simulink model "TCLab_Test_PIL"  (R2026a)
settings: Solver=FixedStepDiscrete  StopTime=t_final  FixedStep=Ts
InitFcn:
  | A8_init_TCLab_SIMC
undefined symbols (not defined in the file): den_Gp_d, dspblkCoreblockFVToolHelper, gcbh, N_delay, num_Gp_d, T_amb, T_ref, Ts
settings Model: SILPILSystemUnderTest=refmodels  Creator=jguerrero  LastModifiedBy=jordy

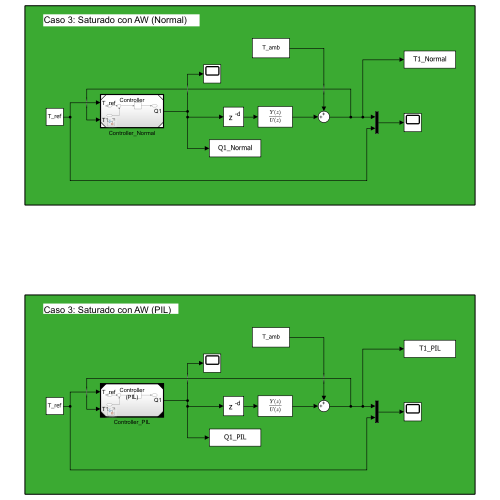
[thumbnail: Simulink's stored preview of the top-level diagram]
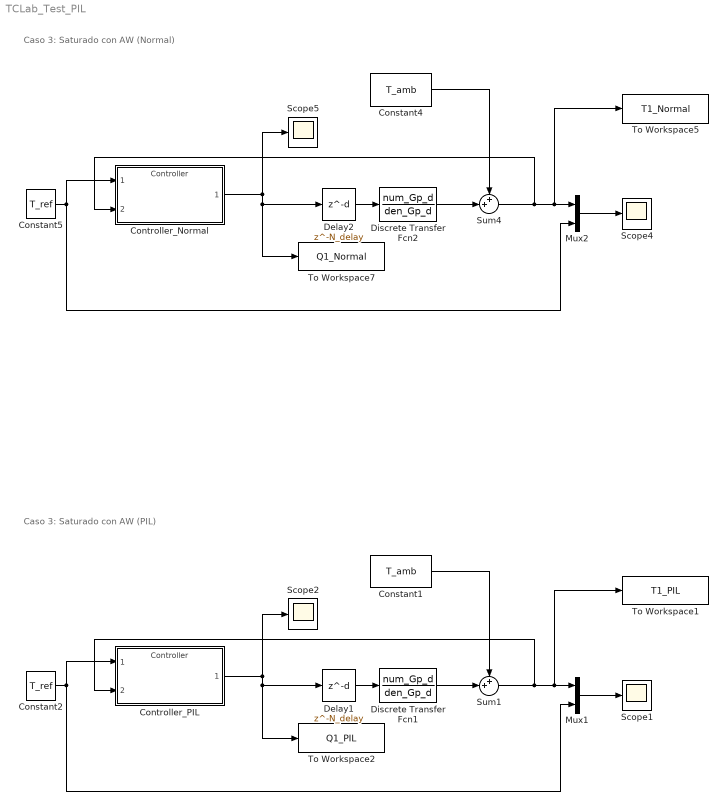
== system TCLab_Test_PIL ==
  note: Caso 3: Saturado con AW (Normal)
  note: Caso 3: Saturado con AW (PIL)
  Constant1 : Constant  Value=T_amb  OutDataTypeStr=single  SampleTime=Ts
  Constant2 : Constant  Value=T_ref  OutDataTypeStr=single  SampleTime=Ts
  Constant4 : Constant  Value=T_amb  OutDataTypeStr=single  SampleTime=Ts
  Constant5 : Constant  Value=T_ref  OutDataTypeStr=single  SampleTime=Ts
  Controller_Normal : ModelReference  ModelNameDialog=Controller  SimulationMode=Normal  ModelReferenceVersion=1.20
  Controller_PIL : ModelReference  ModelNameDialog=Controller  SimulationMode=Processor-in-the-loop (PIL)  ModelReferenceVersion=1.20
  Delay1 : Delay  DelayLength=N_delay  SampleTime=Ts
  Delay2 : Delay  DelayLength=N_delay  SampleTime=Ts
  Discrete Transfer Fcn1 : DiscreteTransferFcn  LoadFcn=dspblkCoreblockFVToolHelper(gcbh,'load');  Numerator=num_Gp_d  Denominator=den_Gp_d
      settings: CopyFcn=dspblkCoreblockFVToolHelper(gcbh,'copy');  DeleteFcn=dspblkCoreblockFVToolHelper(gcbh,'close');  ModelCloseFcn=dspblkCoreblockFVToolHelper(gcbh,'close');  PreSaveFcn=dspblkCoreblockFVToolHelper(gcbh,'presave');  PostSaveFcn=dspblkCoreblockFVToolHelper(gcbh,'postsave');  CloseFcn=dspblkCoreblockFVToolHelper(gcbh,'close');
  Discrete Transfer Fcn2 : DiscreteTransferFcn  LoadFcn=dspblkCoreblockFVToolHelper(gcbh,'load');  Numerator=num_Gp_d  Denominator=den_Gp_d
      settings: CopyFcn=dspblkCoreblockFVToolHelper(gcbh,'copy');  DeleteFcn=dspblkCoreblockFVToolHelper(gcbh,'close');  ModelCloseFcn=dspblkCoreblockFVToolHelper(gcbh,'close');  PreSaveFcn=dspblkCoreblockFVToolHelper(gcbh,'presave');  PostSaveFcn=dspblkCoreblockFVToolHelper(gcbh,'postsave');  CloseFcn=dspblkCoreblockFVToolHelper(gcbh,'close');
  Mux1 : Mux  Inputs=2
  Mux2 : Mux  Inputs=2
  Scope{1..2,4..5} (4 alike) : Scope
      Scope1 settings: ActiveDisplayYMinimum=20.625  ActiveDisplayYMaximum=64.375
      Scope2 settings: ActiveDisplayYMinimum=27.921311930843586  ActiveDisplayYMaximum=96.897632007684052
      Scope4 settings: ActiveDisplayYMinimum=20.625  ActiveDisplayYMaximum=64.375  DataLoggingVariableName=ScopeData4
      Scope5 settings: ActiveDisplayYMinimum=27.921311930843586  ActiveDisplayYMaximum=96.897632007684052  DataLoggingVariableName=ScopeData5
  Sum1 : Sum  Inputs=++|  OutDataTypeStr=single  AccumDataTypeStr=single
  Sum4 : Sum  Inputs=++|  OutDataTypeStr=single  AccumDataTypeStr=single
  To Workspace1 : ToWorkspace  VariableName=T1_PIL  SaveFormat=Timeseries  SampleTime=-1
  To Workspace2 : ToWorkspace  VariableName=Q1_PIL  SaveFormat=Timeseries  SampleTime=-1
  To Workspace5 : ToWorkspace  VariableName=T1_Normal  SaveFormat=Timeseries  SampleTime=-1
  To Workspace7 : ToWorkspace  VariableName=Q1_Normal  SaveFormat=Timeseries  SampleTime=-1
  wires:
  Constant4/1 -> Sum4/1
  Sum4/1 -> Controller_Normal/2, Mux2/1, To Workspace5/1
  Delay2/1 -> Discrete Transfer Fcn2/1
  Discrete Transfer Fcn2/1 -> Sum4/2
  Mux2/1 -> Scope4/1
  Constant5/1 -> Controller_Normal/1, Mux2/2
  Controller_Normal/1 -> To Workspace7/1, Delay2/1, Scope5/1
  Mux1/1 -> Scope1/1
  Constant1/1 -> Sum1/1
  Delay1/1 -> Discrete Transfer Fcn1/1
  Controller_PIL/1 -> To Workspace2/1, Delay1/1, Scope2/1
  Constant2/1 -> Controller_PIL/1, Mux1/2
  Discrete Transfer Fcn1/1 -> Sum1/2
  Sum1/1 -> Controller_PIL/2, Mux1/1, To Workspace1/1
